simulink model "Path_Creation"  (R2023a)
settings: Solver=FixedStepDiscrete  StartTime=0.0  StopTime=100  FixedStep=.02  RelTol=1e-3
libraries: drivinglib x2, simulink x1
settings Model: SimulationMode=accelerator  Creator=FIRSTMentor  LastModifiedBy=FIRSTMentor

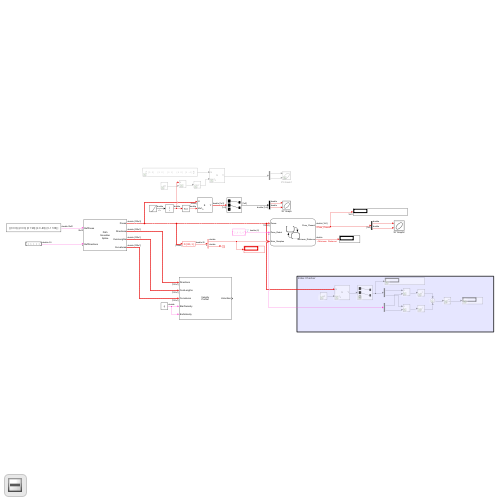
[thumbnail: Simulink's stored preview of the top-level diagram]
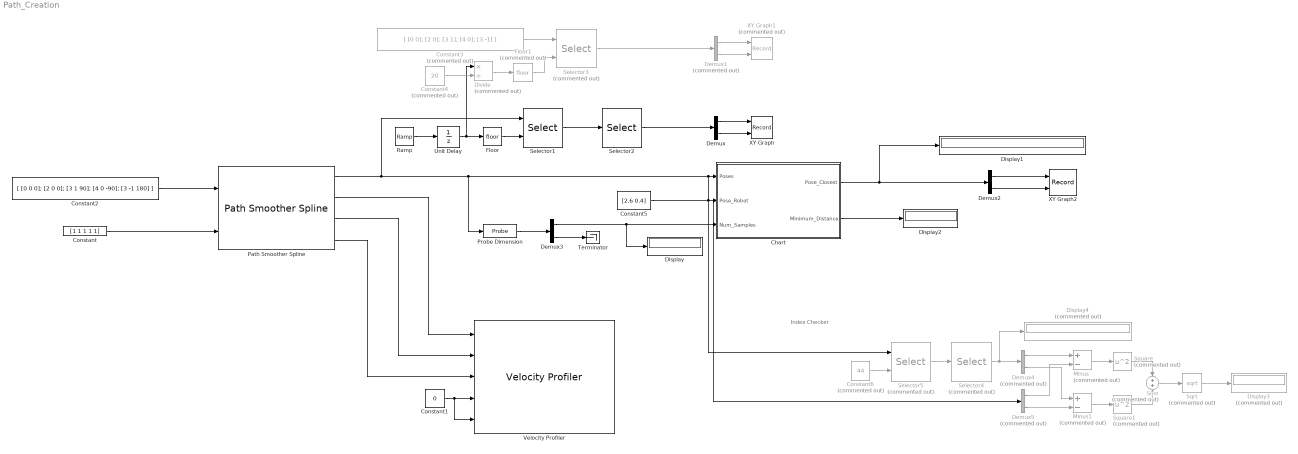
== system Path_Creation ==
  note: Index Checker
  Chart : Stateflow chart  TreatAsAtomicUnit=on
  Constant : Constant  Value=[1 1 1 1 1]
  Constant1 : Constant  Value=0
  Constant2 : Constant  Value=[ [0 0 0]; [2 0 0]; [3 1 90]; [4 0 -90]; [3 -1 180] ]
  Constant3 : Constant  Commented=on  Value=[ [0 0]; [2 0]; [3 1]; [4 0]; [3 -1] ]
  Constant4 : Constant  Commented=on  Value=20
  Constant5 : Constant  Value=[2.6 0.4]
  Constant6 : Constant  Commented=on  Value=44
  Demux : Demux  Outputs=2
  Demux1 : Demux  Commented=on  Outputs=2
  Demux2 : Demux  Outputs=2
  Demux3 : Demux  Outputs=2
  Demux4 : Demux  Commented=on  Outputs=2
  Demux5 : Demux  Commented=on  Outputs=2
  Display : Display
  Display1 : Display
  Display2 : Display
  Display3 : Display  Commented=on
  Display4 : Display  Commented=on
  Divide : Product  Commented=on  Inputs=*/
  Floor : Rounding
  Floor1 : Rounding  Commented=on
  Minus : Sum  Commented=on  Inputs=+-
  Minus1 : Sum  Commented=on  Inputs=+-
  Path Smoother Spline : drivinglib/Path Smoother Spline  NumSmoothPoses=100  MinSeparation=1e-4  SampleTime=0.02  ShowOptionalOutports=on  SimulateUsing=Code generation
  Probe Dimension : Probe  ProbeWidth=off  ProbeSampleTime=off  ProbeComplexSignal=off  ProbeSignalDimensions=on
  Ramp : simulink/Sources/Ramp  slope=1  start=0  InitialOutput=0
  Selector1 : Selector  NumberOfDimensions=2  IndexMode=Zero-based  InputPortWidth=3  IndexOptions=Index vector (port),Select all  Indices=[1 3],1  OutputSizes=1,1
  Selector2 : Selector  IndexMode=Zero-based  InputPortWidth=3  IndexOptions=Index vector (dialog)  Indices=[0 1]  OutputSizes=1
  Selector3 : Selector  Commented=on  NumberOfDimensions=2  IndexMode=Zero-based  InputPortWidth=3  IndexOptions=Index vector (port),Select all  Indices=[1 3],1  OutputSizes=1,1
  Selector4 : Selector  Commented=on  IndexMode=Zero-based  InputPortWidth=3  IndexOptions=Index vector (dialog)  Indices=[0 1]  OutputSizes=1
  Selector5 : Selector  Commented=on  NumberOfDimensions=2  IndexMode=Zero-based  InputPortWidth=3  IndexOptions=Index vector (port),Select all  Indices=[1 3],1  OutputSizes=1,1
  Sqrt : Sqrt  Commented=on
  Square : Math  Commented=on  Operator=square
  Square1 : Math  Commented=on  Operator=square
  Sum : Sum  Commented=on  Inputs=+|+
  Terminator : Terminator
  Unit Delay : UnitDelay  SampleTime=-1  HasFrameUpgradeWarning=on
  Velocity Profiler : drivinglib/Velocity Profiler  MaxLongitudinalAccel=3  MaxLongitudinalDecel=6  MaxSpeed=10  MaxLongitudinalJerk=1  MaxLateralAccel=1  ShowOptionalOutport=off  SampleTime=-1  SimulateUsing=Code generation
  XY Graph : Record  FileSettingsInternal="{\"entries\":[{\"content\":{\"excelSettings\":{\"content\":{},\"type\":\"Streamout.ExcelSettings\"}},\"type\":\"Streamout.FileSettingStorage\",\"uuid\":\"\"}],\"packageUris\":[\"http:\\/\\/schema.mathworks.com\\/mf0\\/streamout_blocks\\/R2020a\"],\"version\":\"1.0\"}"  Layout=[1 1]  SignalsInternal="{\"entries\":[{\"content\":{\"signals\":[{\"content\":{\"blockPath\":[],\"dimensions\":[1,1],\"domain\":\"\",\"lineColor\":\"#a2142f\",\"plots\":[1],\"port\":1,\"sid\":[\"\"],\"signalID\":331,\"signalName\":\"Demux:1\"},\"type\":\"RecordBlkView.Signal\",\"uuid\":\"\"},{\"content\":{\"blockPath\":[],\"dimensions\":[1,1],\"domain\":\"\",\"lineColor\":\"#139fff\",\"plots\":[1],\"port\":2,\"sid\":[\"\"],\"signalID\":335,\"signalName\":\"Demux:2\"},\"type\":\"RecordBlkView.Signal\",\"uuid\":\"\"}]},\"type\":\"RecordBlkView.InputSignals\",\"uuid\":\"\"}],\"packageUris\":[\"http:\\/\\/schema.mathworks.com\\/mf0\\/streamout_blocks\\/R2020a\"],\"version\":\"1.0\"}"  VisualizationBindings="{\"xyplotplugin\":{\"info\":[{\"series\":[{\"bindingParametersList\":[{\"parameter\":\"X-Axis\",\"signalID\":331,\"signalName\":\"Demux:1\"},{\"parameter\":\"Y-Axis\",\"signalID\":335,\"signalName\":\"Demux:2\"}],\"seriesID\":11827}],\"subplotID\":1}]}}"  CompatibilityTag=XY
  XY Graph1 : Record  Commented=on  FileSettingsInternal="{\"entries\":[{\"content\":{\"excelSettings\":{\"content\":{},\"type\":\"Streamout.ExcelSettings\"}},\"type\":\"Streamout.FileSettingStorage\",\"uuid\":\"\"}],\"packageUris\":[\"http:\\/\\/schema.mathworks.com\\/mf0\\/streamout_blocks\\/R2020a\"],\"version\":\"1.0\"}"  Layout=[1 1]  SignalsInternal="{\"entries\":[{\"content\":{},\"type\":\"RecordBlkView.InputSignals\",\"uuid\":\"\"}],\"packageUris\":[\"http:\\/\\/schema.mathworks.com\\/mf0\\/streamout_blocks\\/R2020a\"],\"version\":\"1.0\"}"  VisualizationBindings="{\"sparklinesplugin\":{\"info\":[{\"bindingParametersList\":[],\"subplotID\":1}]}}"  CompatibilityTag=XY
  XY Graph2 : Record  FileSettingsInternal="{\"entries\":[{\"content\":{\"excelSettings\":{\"content\":{},\"type\":\"Streamout.ExcelSettings\"}},\"type\":\"Streamout.FileSettingStorage\",\"uuid\":\"\"}],\"packageUris\":[\"http:\\/\\/schema.mathworks.com\\/mf0\\/streamout_blocks\\/R2020a\"],\"version\":\"1.0\"}"  Layout=[1 1]  SignalsInternal="{\"entries\":[{\"content\":{\"signals\":[{\"content\":{\"blockPath\":[],\"dimensions\":[1,1],\"domain\":\"\",\"lineColor\":\"#a2142f\",\"plots\":[1],\"port\":1,\"sid\":[\"\"],\"signalID\":339,\"signalName\":\"Demux2:1\"},\"type\":\"RecordBlkView.Signal\",\"uuid\":\"\"},{\"content\":{\"blockPath\":[],\"dimensions\":[1,1],\"domain\":\"\",\"lineColor\":\"#139fff\",\"plots\":[1],\"port\":2,\"sid\":[\"\"],\"signalID\":343,\"signalName\":\"Demux2:2\"},\"type\":\"RecordBlkView.Signal\",\"uuid\":\"\"}]},\"type\":\"RecordBlkView.InputSignals\",\"uuid\":\"\"}],\"packageUris\":[\"http:\\/\\/schema.mathworks.com\\/mf0\\/streamout_blocks\\/R2020a\"],\"version\":\"1.0\"}"  VisualizationBindings="{\"xyplotplugin\":{\"info\":[{\"series\":[{\"bindingParametersList\":[{\"parameter\":\"X-Axis\",\"signalID\":339,\"signalName\":\"Demux2:1\"},{\"parameter\":\"Y-Axis\",\"signalID\":343,\"signalName\":\"Demux2:2\"}],\"seriesID\":61170}],\"subplotID\":1}]}}"  CompatibilityTag=XY
  wires:
  Constant/1 -> Path Smoother Spline/2
  Constant1/1 -> Velocity Profiler/5, Velocity Profiler/4
  Constant2/1 -> Path Smoother Spline/1
  Path Smoother Spline/2 -> Velocity Profiler/1
  Path Smoother Spline/3 -> Velocity Profiler/2
  Path Smoother Spline/4 -> Velocity Profiler/3
  Selector1/1 -> Selector2/1
  Ramp/1 -> Unit Delay/1
  Floor/1 -> Selector1/2
  Selector2/1 -> Demux/1
  Demux/2 -> XY Graph/2
  Demux/1 -> XY Graph/1
  Unit Delay/1 -> Divide/1, Floor/1
  Constant3/1 -> Selector3/1
  Selector3/1 -> Demux1/1
  Demux1/1 -> XY Graph1/1
  Demux1/2 -> XY Graph1/2
  Divide/1 -> Floor1/1
  Floor1/1 -> Selector3/2
  Constant4/1 -> Divide/2
  Constant5/1 -> Demux5/1, Chart/2(Pose_Robot)
  Path Smoother Spline/1 -> Selector1/1, Probe Dimension/1, Selector5/1, Chart/1(Poses)
  Probe Dimension/1 -> Demux3/1
  Demux3/1 -> Display/1, Chart/3(Num_Samples)
  Demux3/2 -> Terminator/1
  Chart/1(Pose_Closest) -> Demux2/1, Display1/1
  Chart/2(Minimum_Distance) -> Display2/1
  Demux2/1 -> XY Graph2/1
  Demux2/2 -> XY Graph2/2
  Square/1 -> Sum/1
  Square1/1 -> Sum/2
  Sum/1 -> Sqrt/1
  Minus1/1 -> Square1/1
  Minus/1 -> Square/1
  Selector4/1 -> Display4/1, Demux4/1
  Demux4/1 -> Minus/1
  Demux5/1 -> Minus/2
  Demux4/2 -> Minus1/1
  Demux5/2 -> Minus1/2
  Selector5/1 -> Selector4/1
  Constant6/1 -> Selector5/2
  Sqrt/1 -> Display3/1

== stateflow chart Path_Creation/Chart ==
  (default) -> (junction 2) : {
      | Index_Closest = 1;
      | Minimum_Sum_Squares = (Poses(Index_Closest, 1) - Pose_Robot(1))^2 + (Poses(Index_Closest, 2) - Pose_Robot(2))^2;
      | index=2;
      | }
  (junction 29) -> (junction 2)
  (junction 28) -> (junction 29)
  (junction 2) -> (junction 23) : {
      | Current_Sum_Squares = (Poses(index, 1) - Pose_Robot(1))^2 + (Poses(index, 2) - Pose_Robot(2))^2;
      | }
  (junction 23) -> (junction 19) [order 1] : [Current_Sum_Squares <= Minimum_Sum_Squares]
  (junction 23) -> (junction 4) [order 2]
  (junction 19) -> (junction 32) : {
      | Minimum_Sum_Squares = Current_Sum_Squares;
      | Index_Closest = index;
      | }
  (junction 4) -> (junction 28) [order 1] : [index < Num_Samples]
      | {index=index+1;}
  (junction 32) -> (junction 4)
  (junction 4) -> (junction 12) [order 2] : {
      | Minimum_Distance = sqrt(Minimum_Sum_Squares);
      | Pose_Closest = Poses(Index_Closest, 1:2);
      | }
  data: Poses input size=100,3; index local; Pose_Closest output double size=1,2; Pose_Robot input; Num_Samples input; Current_Sum_Squares local size=1; Minimum_Sum_Squares local; Minimum_Distance output; Index_Closest local
